simulink model "tst5"  (R2024b)
settings: Solver=ode45  StartTime=0.0  StopTime=10  FixedStep=0.001  RelTol=1e-3
settings Model: Creator=LENOVO  LastModifiedBy=LENOVO

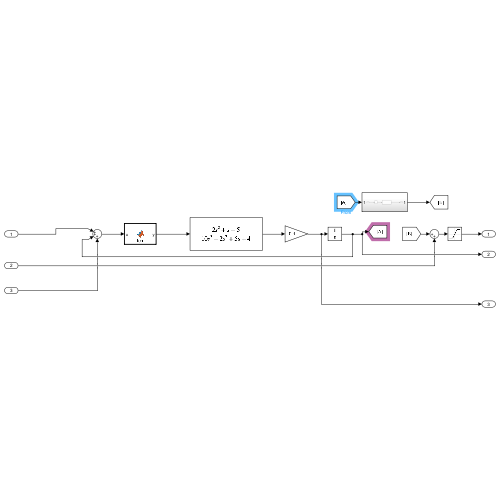
[thumbnail: Simulink's stored preview of the top-level diagram]
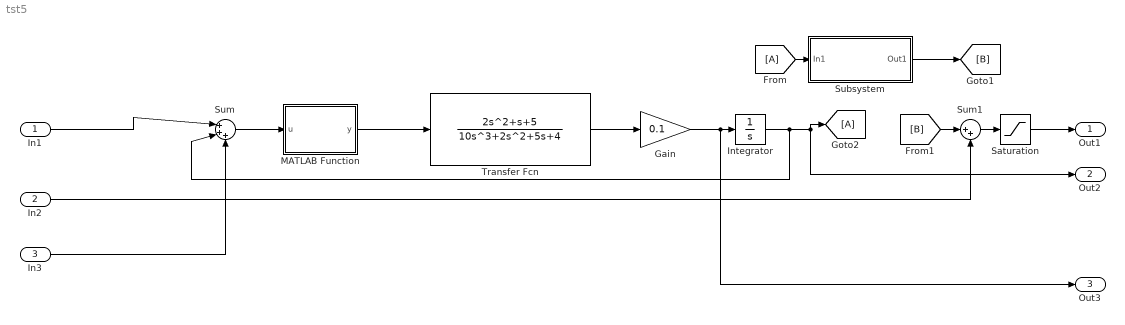
== system tst5 ==
  In1 : Inport
  In2 : Inport  Port=2
  In3 : Inport  Port=3
  From : From
  Gain : Gain  Gain=0.1
  Goto2 : Goto
  Integrator : Integrator  InitialCondition=1
  MATLAB Function : MATLAB Function  TreatAsAtomicUnit=on
  Saturation : Saturate
  Subsystem : Subsystem
  Sum : Sum  Inputs=|+++
  Sum1 : Sum  Inputs=|++
  Transfer Fcn : TransferFcn  Numerator=[2 1 5]  Denominator=[10 2 5 4]
  Out1 : Outport
  Out2 : Outport  Port=2
  Out3 : Outport  Port=3
  wires:
  Integrator/1 -> Sum/2, Goto2/1, Out2/1
  Transfer Fcn/1 -> Gain/1
  Sum/1 -> MATLAB Function/1(u)
  [B] -> Sum1/1
  In2/1 -> Sum1/2
  Sum1/1 -> Saturation/1
  In1/1 -> Sum/1
  Gain/1 -> Out3/1, Integrator/1
  MATLAB Function/1(y) -> Transfer Fcn/1
  In3/1 -> Sum/3
  Saturation/1 -> Out1/1
  From/1 -> Subsystem/1(In1)
  Subsystem/1(Out1) -> [B]

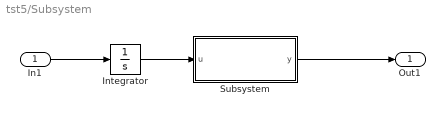
== system tst5/Subsystem ==
  In1 : Inport
  Integrator : Integrator
  Subsystem : Subsystem
  Out1 : Outport
  wires:
  In1/1 -> Integrator/1
  Subsystem/1(y) -> Out1/1
  Integrator/1 -> Subsystem/1(u)

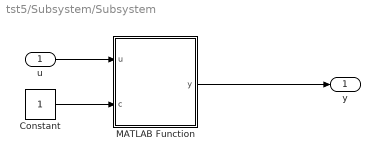
== system tst5/Subsystem/Subsystem ==
  u : Inport
  Constant : Constant
  MATLAB Function : MATLAB Function  TreatAsAtomicUnit=on
  y : Outport
  wires:
  Constant/1 -> MATLAB Function/2(c)
  u/1 -> MATLAB Function/1(u)
  MATLAB Function/1(y) -> y/1

== matlab function tst5/Subsystem/Subsystem/MATLAB Function ==
  data: u input; y output; c input
function y = fcn(u,c)

if u >= 1
    y = 2*u + c;
else
    y = c - u;
end

== matlab function tst5/MATLAB Function ==
  data: u input; y output
function y = fcn(u)
m = 0.1;

y = m*u;
